simulink model "Fourteen_bus_simscape_V1o1"  (R2026a)
settings: Solver=ode23t  StopTime=12  FixedStep=0.2  RelTol=1e-2  AbsTol=1e-2  EnableMultiTasking=on
libraries: ee_lib x92, nesl_utility x64, fl_lib x25, eeRmsMeasurement x18, slpidlib x5, eeSmGovernor x2, elec_conv_HighZElecRef x1
(part 1 of 3)
settings Model: Creator=Bharath  LastModifiedBy=Mudassir
settings SolverCC: MaxConsecutiveMinStep=auto  ZeroCrossControl=DisableAll
settings DataIOCC: SignalLoggingSaveFormat=ModelDataLogs
settings DebuggingCC: SaveWithParameterizedLinksMsg=none  UnderspecifiedInitializationDetection=Classic
settings HardwareCC: ProdHWDeviceType=32-bit Generic
settings GRTTargetCC: CombineOutputUpdateFcns=off  GRTInterface=on
settings SimscapeCC: SimscapeNormalizeSystem=off  SimscapeLogType=none  SimscapeLogDataHistory=5000.0

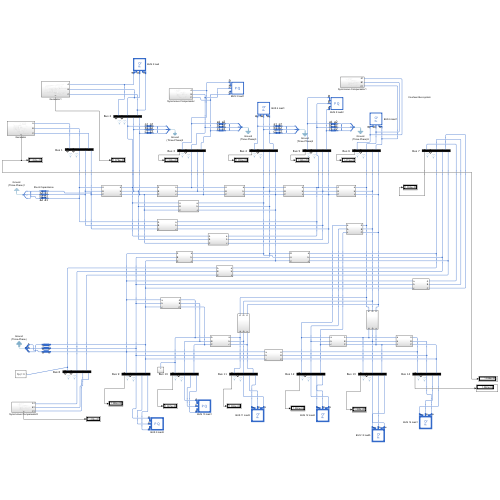
[thumbnail: Simulink's stored preview of the top-level diagram]
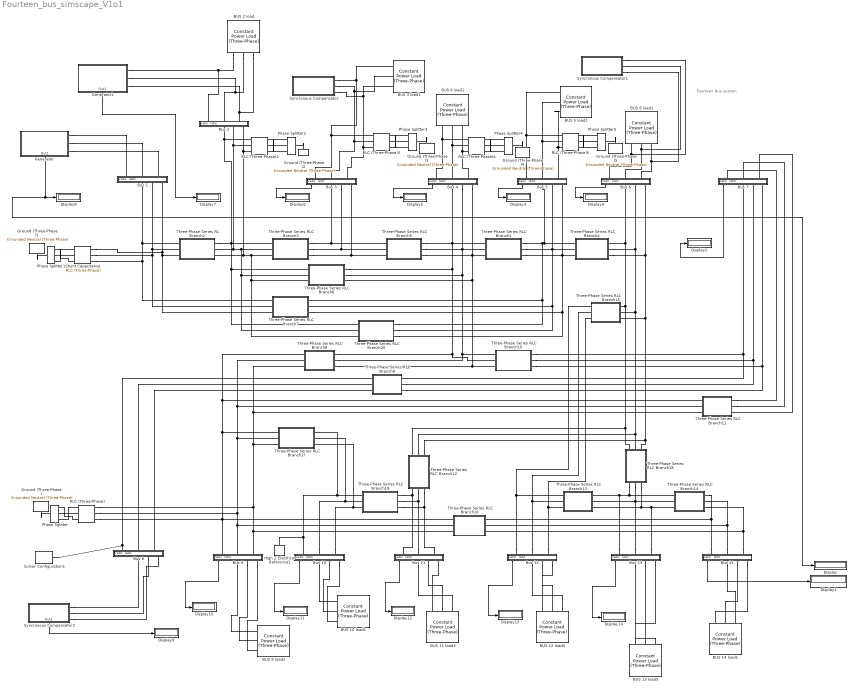
== system Fourteen_bus_simscape_V1o1 ==
  note: Fourteen Bus system
  BUS 10 load1 : ee_lib/Passive/Constant Power Load (Three-Phase)  port_option=ee.enum.threePhasePort.expanded  FRated=60 Hz  active_power=9.0e6 W  reactive_power=5.8e6 A*V  Vline_rms_min=92.4e3 V  tau=0.01 s  Vline_rms_ini=132e3 V  Vang_ini=0 deg  gmin=1e-6 S
  BUS 11 load3 : ee_lib/Passive/Constant Power Load (Three-Phase)  port_option=ee.enum.threePhasePort.expanded  FRated=60 Hz  active_power=3.5e6 W  reactive_power=1.8e6 A*V  Vline_rms_min=92.4e3 V  tau=0.01 s  Vline_rms_ini=132e3 V  Vang_ini=0 deg  gmin=1e-6 S
  BUS 12 load4 : ee_lib/Passive/Constant Power Load (Three-Phase)  port_option=ee.enum.threePhasePort.expanded  FRated=60 Hz  active_power=6.1e6 W  reactive_power=1.6e6 A*V  Vline_rms_min=92.4e3 V  tau=0.01 s  Vline_rms_ini=132e3 V  Vang_ini=0 deg  gmin=1e-6 S
  BUS 13 load5 : ee_lib/Passive/Constant Power Load (Three-Phase)  port_option=ee.enum.threePhasePort.expanded  FRated=60 Hz  active_power=13.5e6 W  reactive_power=5.8e6 A*V  Vline_rms_min=92.3e3 V  tau=0.01 s  Vline_rms_ini=132e3 V  Vang_ini=0 deg  gmin=1e-6 S
  BUS 14 load1 : ee_lib/Passive/Constant Power Load (Three-Phase)  port_option=ee.enum.threePhasePort.expanded  FRated=60 Hz  active_power=14.9e6 W  reactive_power=5.0e6 A*V  Vline_rms_min=92.4e3 V  tau=0.01 s  Vline_rms_ini=132e3 V  Vang_ini=0 deg  gmin=1e-6 S
  BUS 2 load : ee_lib/Passive/Constant Power Load (Three-Phase)  port_option=ee.enum.threePhasePort.expanded  FRated=60 Hz  active_power=21.7e6 W  reactive_power=12.7e6 A*V  Vline_rms_min=92.4 V  tau=0.01 s  Vline_rms_ini=132e3 V  Vang_ini=0 deg  gmin=1e-6 S
  BUS 3 load1 : ee_lib/Passive/Constant Power Load (Three-Phase)  port_option=ee.enum.threePhasePort.expanded  FRated=60 Hz  active_power=94.2e6 W  reactive_power=19.0e6 A*V  Vline_rms_min=92.4e3 V  tau=0.01 s  Vline_rms_ini=132e3 V  Vang_ini=0 deg  gmin=1e-6 S
  BUS 4 load1 : ee_lib/Passive/Constant Power Load (Three-Phase)  port_option=ee.enum.threePhasePort.expanded  FRated=60 Hz  active_power=47.8e6 W  reactive_power=-3.9e6 A*V  Vline_rms_min=92.4e3 V  tau=0.01 s  Vline_rms_ini=132e3 V  Vang_ini=0 deg  gmin=1e-6 S
  BUS 5 load2 : ee_lib/Passive/Constant Power Load (Three-Phase)  port_option=ee.enum.threePhasePort.expanded  FRated=60 Hz  active_power=7.6e6 W  reactive_power=1.6e6 A*V  Vline_rms_min=92.4e3 V  tau=0.01 s  Vline_rms_ini=132e3 V  Vang_ini=0 deg  gmin=1e-6 S
  BUS 6 load1 : ee_lib/Passive/Constant Power Load (Three-Phase)  port_option=ee.enum.threePhasePort.expanded  FRated=60 Hz  active_power=11.2e6 W  reactive_power=7.5e6 A*V  Vline_rms_min=92.4e3 V  tau=0.01 s  Vline_rms_ini=132e3 V  Vang_ini=0 deg  gmin=1e-6 S
  BUS 9 load2 : ee_lib/Passive/Constant Power Load (Three-Phase)  port_option=ee.enum.threePhasePort.expanded  FRated=60 Hz  active_power=29.5e6 W  reactive_power=16.6e6 A*V  Vline_rms_min=92.4e3 V  tau=0.01 s  Vline_rms_ini=132e3 V  Vang_ini=0 deg  gmin=1e-6 S
  "Bus 1 " : Subsystem
  "Bus 10 " : Subsystem
  "Bus 11 " : Subsystem
  "Bus 12 " : Subsystem
  "Bus 13 " : Subsystem
  "Bus 14 " : Subsystem
  "Bus 2 " : Subsystem
  "Bus 3 " : Subsystem
  "Bus 4 " : Subsystem
  "Bus 5 " : Subsystem
  "Bus 6 " : Subsystem
  "Bus 7 " : Subsystem
  "Bus 8 " : Subsystem
  "Bus 9 " : Subsystem
  Display{,1..14} (15 alike) : Display
  Generator : Subsystem
      settings: PortSchema="{\"entries\":[{\"content\":{\"sides\":[{\"content\":{},\"type\":\"ConnectorPlacement.EquallySpacedRectSide\",\"uuid\":\"dad8709b-30c0-4090-88e1-ec810a18cf3f\"},{\"content\":{\"connectorIds\":[\"RConn1\",\"RConn2\",\"RConn3\"],\"side\":\"RIGHT\"},\"type\":\"ConnectorPlacement.EquallySpacedRectSide\",\"uuid\":\"92b3fce1-089d-4b63-9622-725cf932acc2\"},{\"content\":{\"side\":\"TOP\"},\"type\":\"ConnectorPlacement.EquallySpacedRectSide\",\"uuid\":\"fda0afc2-97bc-4766-b49e-326dedc200bc\"},{\"content\":{\"connectorIds\":[\"Out1\"],\"side\":\"BOTTOM\"},\"type\":\"ConnectorPlacement.EquallySpacedRectSide\",\"uuid\":\"7b5f0a66-de7c-4105-acc6-abc867d9e61c\"}]},\"type\":\"ConnectorPlacement.EquallySpacedConnector\",\"uuid\":\"4ba6e797-8987-4af2-b0c1-b0b7a69cc685\"}],\"packageUris\":[\"http://schema.mathworks.com/mf0/Connector/R2020b\"],\"version\":\"1.0\"}"
  Generator1 : Subsystem
      settings: PortSchema="{\"entries\":[{\"content\":{\"sides\":[{\"content\":{},\"type\":\"ConnectorPlacement.EquallySpacedRectSide\",\"uuid\":\"dad8709b-30c0-4090-88e1-ec810a18cf3f\"},{\"content\":{\"connectorIds\":[\"RConn1\",\"RConn2\",\"RConn3\"],\"side\":\"RIGHT\"},\"type\":\"ConnectorPlacement.EquallySpacedRectSide\",\"uuid\":\"92b3fce1-089d-4b63-9622-725cf932acc2\"},{\"content\":{\"side\":\"TOP\"},\"type\":\"ConnectorPlacement.EquallySpacedRectSide\",\"uuid\":\"fda0afc2-97bc-4766-b49e-326dedc200bc\"},{\"content\":{\"connectorIds\":[\"Out1\"],\"side\":\"BOTTOM\"},\"type\":\"ConnectorPlacement.EquallySpacedRectSide\",\"uuid\":\"e381a1c8-2bd2-44ff-8304-e9f3baae7e4f\"}]},\"type\":\"ConnectorPlacement.EquallySpacedConnector\",\"uuid\":\"4ba6e797-8987-4af2-b0c1-b0b7a69cc685\"}],\"packageUris\":[\"http://schema.mathworks.com/mf0/Connector/R2020b\"],\"version\":\"1.0\"}"
  Ground (Three-Phase){,1..5} (6 alike) : ee_lib/Connectors & References/Grounded Neutral (Three-Phase)  port_option=ee.enum.threePhasePort.composite
  High Z Electrical Reference1 : elec_conv_HighZElecRef/High Z Electrical Reference  SystemSampleTime=-1  VariantActivationTime=update diagram  EmptyChoice=off  PassThrough=off  PassThroughVariantControl=(default)  EmptyChoiceVariantControl=(default)  AllowFlexibleInterface=on  Latency=0  AutoFrameSizeCalculation=off
  Phase Splitter{,1..5} (6 alike) : ee_lib/Connectors & References/Phase Splitter
  RLC (Three-Phase) : ee_lib/Passive/RLC Assemblies/RLC (Three-Phase)  port_option=ee.enum.threePhasePort.expanded  component_structure=ee.enum.rlc.structure.C  R=1 Ohm  L=1e-3 H  C=2.892e-6 F  R_parasitic=1 Ohm  G_parasitic=0 1/Ohm  IL_specify=off  IL_priority=High  IL=[0, 0, 0] A  IL_nominal_specify=off  IL_nominal_value=1  IL_nominal_unit=A  VC_specify=off  VC_priority=High  VC=[0, 0, 0] V  VC_nominal_specify=off  VC_nominal_value=1  VC_nominal_unit=V
  RLC (Three-Phase)2 : ee_lib/Passive/RLC Assemblies/RLC (Three-Phase)  port_option=ee.enum.threePhasePort.expanded  component_structure=ee.enum.rlc.structure.C  R=1 Ohm  L=1e-3 H  C=1.257e-6 F  R_parasitic=1 Ohm  G_parasitic=0 1/Ohm  IL_specify=off  IL_priority=High  IL=[0, 0, 0] A  IL_nominal_specify=off  IL_nominal_value=1  IL_nominal_unit=A  VC_specify=off  VC_priority=High  VC=[0, 0, 0] V  VC_nominal_specify=off  VC_nominal_value=1  VC_nominal_unit=V
  RLC (Three-Phase)3 : ee_lib/Passive/RLC Assemblies/RLC (Three-Phase)  port_option=ee.enum.threePhasePort.expanded  component_structure=ee.enum.rlc.structure.C  R=1 Ohm  L=1e-3 H  C=5.922e-7 F  R_parasitic=1 Ohm  G_parasitic=0 1/Ohm  IL_specify=off  IL_priority=High  IL=[0, 0, 0] A  IL_nominal_specify=off  IL_nominal_value=1  IL_nominal_unit=A  VC_specify=off  VC_priority=High  VC=[0, 0, 0] V  VC_nominal_specify=off  VC_nominal_value=1  VC_nominal_unit=V
  RLC (Three-Phase)4 : ee_lib/Passive/RLC Assemblies/RLC (Three-Phase)  port_option=ee.enum.threePhasePort.expanded  component_structure=ee.enum.rlc.structure.C  R=1 Ohm  L=1e-3 H  C=5.176e-7 F  R_parasitic=1 Ohm  G_parasitic=0 1/Ohm  IL_specify=off  IL_priority=High  IL=[0, 0, 0] A  IL_nominal_specify=off  IL_nominal_value=1  IL_nominal_unit=A  VC_specify=off  VC_priority=High  VC=[0, 0, 0] V  VC_nominal_specify=off  VC_nominal_value=1  VC_nominal_unit=V
  RLC (Three-Phase)5 : ee_lib/Passive/RLC Assemblies/RLC (Three-Phase)  port_option=ee.enum.threePhasePort.expanded  component_structure=ee.enum.rlc.structure.C  R=1 Ohm  L=1e-3 H  C=6.493e-7 F  R_parasitic=1 Ohm  G_parasitic=0 1/Ohm  IL_specify=off  IL_priority=High  IL=[0, 0, 0] A  IL_nominal_specify=off  IL_nominal_value=1  IL_nominal_unit=A  VC_specify=off  VC_priority=High  VC=[0, 0, 0] V  VC_nominal_specify=off  VC_nominal_value=1  VC_nominal_unit=V
  Shunt Capacitance : ee_lib/Passive/RLC Assemblies/RLC (Three-Phase)  port_option=ee.enum.threePhasePort.expanded  component_structure=ee.enum.rlc.structure.C  R=1 Ohm  L=1e-3 H  C=7.878e-7 F  R_parasitic=1 Ohm  G_parasitic=0 1/Ohm  IL_specify=off  IL_priority=High  IL=[0, 0, 0] A  IL_nominal_specify=off  IL_nominal_value=1  IL_nominal_unit=A  VC_specify=off  VC_priority=High  VC=[0, 0, 0] V  VC_nominal_specify=off  VC_nominal_value=1  VC_nominal_unit=V
  Solver Configuration1 : nesl_utility/Solver Configuration  PhysicalDomain=network_engine_domain  SubClassName=solver  LeftPortType=input  RightPortType=generic  Tones=[]  Harmonics=[]  SimulateNoise=off  Profile=off  UseLocalSampling=off  EnableSwitchedLinearOptims=on  FrequencyDomain=off  UseCCode=off  RelTol=0.001  AbsTol=0.001  MinStep=1e-09  ToWorkspace=off  RevertToSquareIcSolve=off  NumHomotopyIterations=100  PhasorMode=off  PhasorModeNumHarmonics=1  ConsistencySolver=NEWTON_XTOL_AFTER_FTOL  CanonicalOrdering=CANONICAL  OptimizeIntermediates=OPTIMIZED  IndexReductionMethod=DerivativeReplacement  DoDC=off  ResidualTolerance=1e-09  ConsistencyTolSource=GLOBAL  ConsistencyAbsTol=0.001  ConsistencyRelTol=0.001  ConsistencyTolFactor=0.001  UseLocalSolver=off  LocalSolverChoice=NE_BACKWARD_EULER_ADVANCER  ResolveIndetEquations=on  FunctionEvalNumThread=1  LocalSolverSampleTime=0.001  DoFixedCost=off  MaxNonlinIter=3  MaxModeIter=2  ComputeImpulses=off  ImpulseIterations=2  LinearAlgebra=auto  LinearAlgebraNumThread=0  EquationFormulation=NE_TIME_EF  DelaysMemoryBudget=1024  AutomaticFiltering=on  FilteringTimeConstant=0.001  PartitionStorageMethod=AS_NEEDED  PartitionMemoryBudget=1024  PartitionMethod=ROBUST  MultibodyUseLocalSolver=off  MultibodyLocalSolverChoice=ODE1  MultibodyLocalSolverSampleTime=0.001
  Syncronous Compensator : Subsystem
  Syncronous Compensator1 : Subsystem
  Syncronous Compensator2 : Subsystem
      settings: PortSchema="{\"entries\":[{\"content\":{\"sides\":[{\"content\":{},\"type\":\"ConnectorPlacement.EquallySpacedRectSide\",\"uuid\":\"dad8709b-30c0-4090-88e1-ec810a18cf3f\"},{\"content\":{\"connectorIds\":[\"RConn1\",\"RConn2\",\"RConn3\"],\"side\":\"RIGHT\"},\"type\":\"ConnectorPlacement.EquallySpacedRectSide\",\"uuid\":\"92b3fce1-089d-4b63-9622-725cf932acc2\"},{\"content\":{\"side\":\"TOP\"},\"type\":\"ConnectorPlacement.EquallySpacedRectSide\",\"uuid\":\"fda0afc2-97bc-4766-b49e-326dedc200bc\"},{\"content\":{\"connectorIds\":[\"Out1\"],\"side\":\"BOTTOM\"},\"type\":\"ConnectorPlacement.EquallySpacedRectSide\",\"uuid\":\"87e71bf6-f82f-4acd-82d9-e7a3dc4e74e7\"}]},\"type\":\"ConnectorPlacement.EquallySpacedConnector\",\"uuid\":\"4ba6e797-8987-4af2-b0c1-b0b7a69cc685\"}],\"packageUris\":[\"http://schema.mathworks.com/mf0/Connector/R2020b\"],\"version\":\"1.0\"}"
  Three-Phase Series RL Branch2 : Subsystem
      settings: AttributesFormatString=\n
  Three-Phase Series RLC Branch1 : Subsystem
      settings: AttributesFormatString=\n
  Three-Phase Series RLC Branch10 : Subsystem
      settings: AttributesFormatString=\n
  Three-Phase Series RLC Branch11 : Subsystem
      settings: AttributesFormatString=\n
  Three-Phase Series RLC Branch12 : Subsystem
      settings: AttributesFormatString=\n
  Three-Phase Series RLC Branch13 : Subsystem
      settings: AttributesFormatString=\n
  Three-Phase Series RLC Branch14 : Subsystem
      settings: AttributesFormatString=\n
  Three-Phase Series RLC Branch15 : Subsystem
      settings: AttributesFormatString=\n
  Three-Phase Series RLC Branch16 : Subsystem
      settings: AttributesFormatString=\n
  Three-Phase Series RLC Branch17 : Subsystem
      settings: AttributesFormatString=\n
  Three-Phase Series RLC Branch18 : Subsystem
      settings: AttributesFormatString=\n
  Three-Phase Series RLC Branch19 : Subsystem
      settings: AttributesFormatString=\n
  Three-Phase Series RLC Branch20 : Subsystem
      settings: AttributesFormatString=\n
  Three-Phase Series RLC Branch3 : Subsystem
      settings: AttributesFormatString=\n
  Three-Phase Series RLC Branch4 : Subsystem
      settings: AttributesFormatString=\n
  Three-Phase Series RLC Branch5 : Subsystem
      settings: AttributesFormatString=\n
  Three-Phase Series RLC Branch6 : Subsystem
      settings: AttributesFormatString=\n
  Three-Phase Series RLC Branch7 : Subsystem
      settings: AttributesFormatString=\n
  Three-Phase Series RLC Branch8 : Subsystem
      settings: AttributesFormatString=\n
  Three-Phase Series RLC Branch9 : Subsystem
      settings: AttributesFormatString=\n
  wires:
  "Bus 7 "/1(Vabc) -> Display2/1
  "Bus 5 "/1(Vabc) -> Display3/1
  "Bus 6 "/1(Vabc) -> Display4/1
  "Bus 4 "/1(Vabc) -> Display5/1
  "Bus 3 "/1(Vabc) -> Display6/1
  Generator1/1(Out1) -> Display7/1
  Generator/1(Out1) -> Display/1, Display8/1
  Syncronous Compensator2/1(Out1) -> Display9/1
  "Bus 9 "/1(Vabc) -> Display10/1
  "Bus 10 "/1(Vabc) -> Display11/1
  "Bus 11 "/1(Vabc) -> Display12/1
  "Bus 12 "/1(Vabc) -> Display13/1
  "Bus 13 "/1(Vabc) -> Display14/1
  "Bus 14 "/1(Vabc) -> Display1/1
  connections:
  "Bus 9 "/LConn3 -- Three-Phase Series RLC Branch16/RConn3 -- RLC (Three-Phase)/LConn3 -- Three-Phase Series RLC Branch17/RConn3 -- Three-Phase Series RLC Branch11/RConn3 -- Three-Phase Series RLC Branch8/LConn3
  "Bus 9 "/LConn2 -- Three-Phase Series RLC Branch16/RConn2 -- RLC (Three-Phase)/LConn2 -- Three-Phase Series RLC Branch17/RConn2 -- Three-Phase Series RLC Branch11/RConn2 -- Three-Phase Series RLC Branch8/LConn2
  "Bus 9 "/LConn1 -- RLC (Three-Phase)/LConn1 -- Three-Phase Series RLC Branch16/RConn1 -- Three-Phase Series RLC Branch17/RConn1 -- Three-Phase Series RLC Branch11/RConn1 -- Three-Phase Series RLC Branch8/LConn1
  "Bus 7 "/RConn3 -- Three-Phase Series RLC Branch10/RConn3 -- Three-Phase Series RLC Branch9/RConn3
  "Bus 7 "/RConn2 -- Three-Phase Series RLC Branch10/RConn2 -- Three-Phase Series RLC Branch9/RConn2
  "Bus 7 "/RConn1 -- Three-Phase Series RLC Branch10/RConn1 -- Three-Phase Series RLC Branch9/RConn1
  "Bus 6 "/RConn3 -- Three-Phase Series RLC Branch4/RConn3 -- Three-Phase Series RLC Branch18/LConn3 -- Three-Phase Series RLC Branch12/LConn3 -- Three-Phase Series RLC Branch15/LConn3
  "Bus 6 "/RConn2 -- Three-Phase Series RLC Branch15/LConn2 -- Three-Phase Series RLC Branch18/LConn2 -- Three-Phase Series RLC Branch12/LConn2 -- Three-Phase Series RLC Branch4/RConn2
  "Bus 6 "/RConn1 -- Three-Phase Series RLC Branch18/LConn1 -- Three-Phase Series RLC Branch12/LConn1 -- Three-Phase Series RLC Branch15/LConn1 -- Three-Phase Series RLC Branch4/RConn1
  "Bus 5 "/RConn3 -- Three-Phase Series RLC Branch1/RConn3 -- Three-Phase Series RLC Branch20/RConn3 -- Three-Phase Series RLC Branch7/RConn3 -- Three-Phase Series RLC Branch4/LConn3
  "Bus 5 "/RConn2 -- Three-Phase Series RLC Branch1/RConn2 -- Three-Phase Series RLC Branch20/RConn2 -- Three-Phase Series RLC Branch7/RConn2 -- Three-Phase Series RLC Branch4/LConn2
  "Bus 5 "/RConn1 -- Three-Phase Series RLC Branch1/RConn1 -- Three-Phase Series RLC Branch20/RConn1 -- Three-Phase Series RLC Branch7/RConn1 -- Three-Phase Series RLC Branch4/LConn1
  "Bus 3 "/RConn2 -- Three-Phase Series RLC Branch5/LConn2 -- Three-Phase Series RLC Branch3/RConn2
  "Bus 3 "/RConn1 -- Three-Phase Series RLC Branch5/LConn1 -- Three-Phase Series RLC Branch3/RConn1
  Three-Phase Series RLC Branch20/LConn3 -- Three-Phase Series RLC Branch6/LConn3 -- Three-Phase Series RLC Branch3/LConn3 -- Three-Phase Series RL Branch2/RConn3 -- RLC (Three-Phase)2/LConn3 -- "Bus 2 "/RConn3
  Three-Phase Series RLC Branch3/LConn2 -- Three-Phase Series RLC Branch20/LConn2 -- Three-Phase Series RLC Branch6/LConn2 -- Three-Phase Series RL Branch2/RConn2 -- RLC (Three-Phase)2/LConn2 -- "Bus 2 "/RConn2
  Three-Phase Series RLC Branch3/LConn1 -- Three-Phase Series RLC Branch20/LConn1 -- Three-Phase Series RLC Branch6/LConn1 -- Three-Phase Series RL Branch2/RConn1 -- RLC (Three-Phase)2/LConn1 -- "Bus 2 "/RConn1
  BUS 2 load/LConn2 -- Generator1/RConn2 -- "Bus 2 "/LConn2
  BUS 2 load/LConn1 -- Generator1/RConn1 -- "Bus 2 "/LConn1
  "Bus 14 "/LConn3 -- Three-Phase Series RLC Branch14/LConn3 -- Three-Phase Series RLC Branch16/LConn3
  "Bus 14 "/LConn2 -- Three-Phase Series RLC Branch14/LConn2 -- Three-Phase Series RLC Branch16/LConn2
  "Bus 14 "/LConn1 -- Three-Phase Series RLC Branch14/LConn1 -- Three-Phase Series RLC Branch16/LConn1
  "Bus 13 "/LConn3 -- Three-Phase Series RLC Branch18/RConn3 -- Three-Phase Series RLC Branch13/LConn3 -- Three-Phase Series RLC Branch14/RConn3
  "Bus 13 "/LConn2 -- Three-Phase Series RLC Branch18/RConn2 -- Three-Phase Series RLC Branch14/RConn2 -- Three-Phase Series RLC Branch13/LConn2
  "Bus 13 "/LConn1 -- Three-Phase Series RLC Branch18/RConn1 -- Three-Phase Series RLC Branch14/RConn1 -- Three-Phase Series RLC Branch13/LConn1
  "Bus 12 "/LConn3 -- Three-Phase Series RLC Branch13/RConn3 -- Three-Phase Series RLC Branch15/RConn3
  "Bus 12 "/LConn2 -- Three-Phase Series RLC Branch13/RConn2 -- Three-Phase Series RLC Branch15/RConn2
  "Bus 12 "/LConn1 -- Three-Phase Series RLC Branch13/RConn1 -- Three-Phase Series RLC Branch15/RConn1
  "Bus 11 "/LConn3 -- Three-Phase Series RLC Branch12/RConn3 -- Three-Phase Series RLC Branch19/RConn3
  "Bus 11 "/LConn2 -- Three-Phase Series RLC Branch12/RConn2 -- Three-Phase Series RLC Branch19/RConn2
  "Bus 11 "/LConn1 -- Three-Phase Series RLC Branch12/RConn1 -- Three-Phase Series RLC Branch19/RConn1
  "Bus 10 "/LConn3 -- Three-Phase Series RLC Branch17/LConn3 -- Three-Phase Series RLC Branch19/LConn3
  "Bus 10 "/LConn2 -- Three-Phase Series RLC Branch17/LConn2 -- Three-Phase Series RLC Branch19/LConn2
  Three-Phase Series RLC Branch17/LConn1 -- Three-Phase Series RLC Branch19/LConn1 -- "Bus 10 "/LConn1 -- High Z Electrical Reference1/LConn1
  Three-Phase Series RL Branch2/LConn3 -- Three-Phase Series RLC Branch7/LConn3 -- "Bus 1 "/RConn3 -- Shunt Capacitance/LConn3
  "Bus 1 "/RConn2 -- Three-Phase Series RL Branch2/LConn2 -- Shunt Capacitance/LConn2 -- Three-Phase Series RLC Branch7/LConn2
  "Bus 1 "/RConn1 -- Three-Phase Series RL Branch2/LConn1 -- Shunt Capacitance/LConn1 -- Three-Phase Series RLC Branch7/LConn1
  "Bus 4 "/LConn3 -- RLC (Three-Phase)4/LConn3 -- BUS 4 load1/LConn3
  Syncronous Compensator2/RConn3 -- "Bus 8 "/RConn3
  Syncronous Compensator2/RConn2 -- "Bus 8 "/RConn2
  Syncronous Compensator2/RConn1 -- "Bus 8 "/RConn1
  "Bus 9 "/RConn2 -- BUS 9 load2/LConn2
  "Bus 9 "/RConn1 -- BUS 9 load2/LConn1
  "Bus 9 "/RConn3 -- BUS 9 load2/LConn3
  "Bus 4 "/LConn2 -- RLC (Three-Phase)4/LConn2 -- BUS 4 load1/LConn2
  BUS 5 load2/LConn1 -- RLC (Three-Phase)5/LConn1 -- "Bus 5 "/LConn1
  BUS 5 load2/LConn3 -- RLC (Three-Phase)5/LConn3 -- "Bus 5 "/LConn3
  "Bus 7 "/LConn3 -- Three-Phase Series RLC Branch11/LConn3
  BUS 5 load2/LConn2 -- "Bus 5 "/LConn2 -- RLC (Three-Phase)5/LConn2
  "Bus 14 "/RConn3 -- BUS 14 load1/LConn3
  "Bus 14 "/RConn2 -- BUS 14 load1/LConn2
  "Bus 14 "/RConn1 -- BUS 14 load1/LConn1
  "Bus 13 "/RConn3 -- BUS 13 load5/LConn3
  "Bus 13 "/RConn2 -- BUS 13 load5/LConn2
  "Bus 13 "/RConn1 -- BUS 13 load5/LConn1
  "Bus 12 "/RConn3 -- BUS 12 load4/LConn3
  "Bus 12 "/RConn2 -- BUS 12 load4/LConn2
  "Bus 12 "/RConn1 -- BUS 12 load4/LConn1
  "Bus 11 "/RConn3 -- BUS 11 load3/LConn3
  "Bus 11 "/RConn2 -- BUS 11 load3/LConn2
  "Bus 11 "/RConn1 -- BUS 11 load3/LConn1
  "Bus 10 "/RConn3 -- BUS 10 load1/LConn3
  "Bus 10 "/RConn2 -- BUS 10 load1/LConn2
  "Bus 10 "/RConn1 -- BUS 10 load1/LConn1
  BUS 2 load/LConn3 -- Generator1/RConn3 -- "Bus 2 "/LConn3
  "Bus 8 "/LConn1 -- Three-Phase Series RLC Branch9/LConn1 -- Solver Configuration1/RConn1
  Three-Phase Series RLC Branch9/LConn2 -- "Bus 8 "/LConn2
  Three-Phase Series RLC Branch9/LConn3 -- "Bus 8 "/LConn3
  "Bus 4 "/LConn1 -- RLC (Three-Phase)4/LConn1 -- BUS 4 load1/LConn1
  Three-Phase Series RLC Branch11/LConn2 -- "Bus 7 "/LConn2
  Three-Phase Series RLC Branch11/LConn1 -- "Bus 7 "/LConn1
  Syncronous Compensator/RConn2 -- BUS 3 load1/LConn2 -- "Bus 3 "/LConn2 -- RLC (Three-Phase)3/LConn2
  Syncronous Compensator/RConn1 -- BUS 3 load1/LConn1 -- RLC (Three-Phase)3/LConn1 -- "Bus 3 "/LConn1
  Syncronous Compensator/RConn3 -- BUS 3 load1/LConn3 -- RLC (Three-Phase)3/LConn3 -- "Bus 3 "/LConn3
  "Bus 6 "/LConn2 -- Syncronous Compensator1/RConn2 -- BUS 6 load1/LConn2
  "Bus 6 "/LConn1 -- Syncronous Compensator1/RConn1 -- BUS 6 load1/LConn1
  "Bus 6 "/LConn3 -- Syncronous Compensator1/RConn3 -- BUS 6 load1/LConn3
  "Bus 4 "/RConn3 -- Three-Phase Series RLC Branch1/LConn3 -- Three-Phase Series RLC Branch5/RConn3 -- Three-Phase Series RLC Branch6/RConn3 -- Three-Phase Series RLC Branch10/LConn3 -- Three-Phase Series RLC Branch8/RConn3
  "Bus 4 "/RConn2 -- Three-Phase Series RLC Branch1/LConn2 -- Three-Phase Series RLC Branch6/RConn2 -- Three-Phase Series RLC Branch8/RConn2 -- Three-Phase Series RLC Branch10/LConn1 -- Three-Phase Series RLC Branch5/RConn2
  "Bus 4 "/RConn1 -- Three-Phase Series RLC Branch1/LConn1 -- Three-Phase Series RLC Branch6/RConn1 -- Three-Phase Series RLC Branch10/LConn2 -- Three-Phase Series RLC Branch8/RConn1 -- Three-Phase Series RLC Branch5/RConn1
  "Bus 3 "/RConn3 -- Three-Phase Series RLC Branch5/LConn3 -- Three-Phase Series RLC Branch3/RConn3
  Generator/RConn3 -- "Bus 1 "/LConn3
  Generator/RConn1 -- "Bus 1 "/LConn1
  Generator/RConn2 -- "Bus 1 "/LConn2
  Ground (Three-Phase)/LConn1 -- Phase Splitter/LConn1
  RLC (Three-Phase)/RConn3 -- Phase Splitter/RConn3
  RLC (Three-Phase)/RConn2 -- Phase Splitter/RConn2
  RLC (Three-Phase)/RConn1 -- Phase Splitter/RConn1
  Shunt Capacitance/RConn1 -- Phase Splitter1/RConn1
  Ground (Three-Phase)1/LConn1 -- Phase Splitter1/LConn1
  Shunt Capacitance/RConn3 -- Phase Splitter1/RConn3
  Shunt Capacitance/RConn2 -- Phase Splitter1/RConn2
  RLC (Three-Phase)2/RConn3 -- Phase Splitter2/RConn3
  RLC (Three-Phase)2/RConn2 -- Phase Splitter2/RConn2
  Ground (Three-Phase)2/LConn1 -- Phase Splitter2/LConn1
  RLC (Three-Phase)2/RConn1 -- Phase Splitter2/RConn1
  RLC (Three-Phase)3/RConn3 -- Phase Splitter3/RConn3
  RLC (Three-Phase)3/RConn2 -- Phase Splitter3/RConn2
  Ground (Three-Phase)3/LConn1 -- Phase Splitter3/LConn1
  RLC (Three-Phase)3/RConn1 -- Phase Splitter3/RConn1
  RLC (Three-Phase)4/RConn3 -- Phase Splitter4/RConn3
  RLC (Three-Phase)4/RConn2 -- Phase Splitter4/RConn2
  Ground (Three-Phase)4/LConn1 -- Phase Splitter4/LConn1
  RLC (Three-Phase)4/RConn1 -- Phase Splitter4/RConn1
  RLC (Three-Phase)5/RConn3 -- Phase Splitter5/RConn3
  RLC (Three-Phase)5/RConn2 -- Phase Splitter5/RConn2
  Ground (Three-Phase)5/LConn1 -- Phase Splitter5/LConn1
  RLC (Three-Phase)5/RConn1 -- Phase Splitter5/RConn1

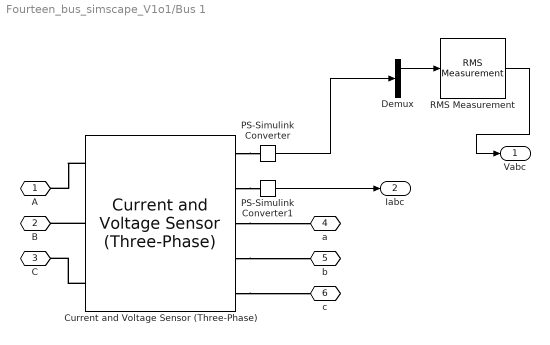
== system Fourteen_bus_simscape_V1o1/Bus 1  ==
  Current and Voltage Sensor (Three-Phase) : ee_lib/Sensors & Transducers/Current and Voltage Sensor (Three-Phase)  port_option=ee.enum.threePhasePort.expanded  vMeasurementType=ee.enum.vmeasurement.ll  outputUnit=ee.enum.unit.si  SRated=100000000 V*A  VRated=0.95 V  I_specify=off  I_priority=None  I=[ 0 0 0 ] A  I_nominal_specify=off  I_nominal_value=1  I_nominal_unit=A  V_specify=off  V_priority=None  V=[ 0 0 0 ] V  V_nominal_specify=off  V_nominal_value=1  V_nominal_unit=V
  Demux : Demux  Outputs=3
  PS-Simulink Converter : nesl_utility/PS-Simulink Converter  PhysicalDomain=network_engine_domain  SubClassName=ps_output  LeftPortType=input  RightPortType=output  PseudoPeriodic=off  Frequencies=[]  VectorFormat=1-D array  Unit=1  AffineConversion=off
  PS-Simulink Converter1 : nesl_utility/PS-Simulink Converter  PhysicalDomain=network_engine_domain  SubClassName=ps_output  LeftPortType=input  RightPortType=output  PseudoPeriodic=off  Frequencies=[]  VectorFormat=1-D array  Unit=1  AffineConversion=off
  RMS Measurement : eeRmsMeasurement/RMS Measurement  LabelModeActiveChoice=Total  F=60  SpecifyHarmonics=off  K=[0 1 2]  Ts=0
      settings: LibrarySourceBlock=|
      | ee_sl_lib/Measurements/RMS
      | Measurement
  A : PMIOPort  Side=Left
  B : PMIOPort  Port=2  Side=Left
  C : PMIOPort  Port=3  Side=Left
  a : PMIOPort  Port=4  Side=Right
  b : PMIOPort  Port=5  Side=Right
  c : PMIOPort  Port=6  Side=Right
  Vabc : Outport  VectorParamsAs1DForOutWhenUnconnected=off
  Iabc : Outport  Port=2  VectorParamsAs1DForOutWhenUnconnected=off
  wires:
  PS-Simulink Converter1/1 -> Iabc/1
  RMS Measurement/1 -> Vabc/1
  Demux/1 -> RMS Measurement/1
  PS-Simulink Converter/1 -> Demux/1
  connections:
  Current and Voltage Sensor (Three-Phase)/RConn1 -- PS-Simulink Converter/LConn1
  Current and Voltage Sensor (Three-Phase)/RConn2 -- PS-Simulink Converter1/LConn1
  Current and Voltage Sensor (Three-Phase)/RConn5 -- c/RConn1
  Current and Voltage Sensor (Three-Phase)/RConn4 -- b/RConn1
  Current and Voltage Sensor (Three-Phase)/RConn3 -- a/RConn1
  Current and Voltage Sensor (Three-Phase)/LConn3 -- C/RConn1
  Current and Voltage Sensor (Three-Phase)/LConn1 -- A/RConn1
  Current and Voltage Sensor (Three-Phase)/LConn2 -- B/RConn1

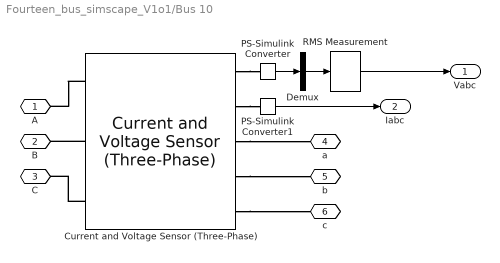
== system Fourteen_bus_simscape_V1o1/Bus 10  ==
  Current and Voltage Sensor (Three-Phase) : ee_lib/Sensors & Transducers/Current and Voltage Sensor (Three-Phase)  port_option=ee.enum.threePhasePort.expanded  vMeasurementType=ee.enum.vmeasurement.ll  outputUnit=ee.enum.unit.si  SRated=100000000 V*A  VRated=0.94 V  I_specify=off  I_priority=None  I=[ 0 0 0 ] A  I_nominal_specify=off  I_nominal_value=1  I_nominal_unit=A  V_specify=off  V_priority=None  V=[ 0 0 0 ] V  V_nominal_specify=off  V_nominal_value=1  V_nominal_unit=V
  Demux : Demux  Outputs=3
  PS-Simulink Converter : nesl_utility/PS-Simulink Converter  PhysicalDomain=network_engine_domain  SubClassName=ps_output  LeftPortType=input  RightPortType=output  PseudoPeriodic=off  Frequencies=[]  VectorFormat=1-D array  Unit=1  AffineConversion=off
  PS-Simulink Converter1 : nesl_utility/PS-Simulink Converter  PhysicalDomain=network_engine_domain  SubClassName=ps_output  LeftPortType=input  RightPortType=output  PseudoPeriodic=off  Frequencies=[]  VectorFormat=1-D array  Unit=1  AffineConversion=off
  RMS Measurement : eeRmsMeasurement/RMS Measurement  LabelModeActiveChoice=Total  F=60  SpecifyHarmonics=off  K=[0 1 2]  Ts=0
      settings: LibrarySourceBlock=|
      | ee_sl_lib/Measurements/RMS
      | Measurement
  A : PMIOPort  Side=Left
  B : PMIOPort  Port=2  Side=Left
  C : PMIOPort  Port=3  Side=Left
  a : PMIOPort  Port=4  Side=Right
  b : PMIOPort  Port=5  Side=Right
  c : PMIOPort  Port=6  Side=Right
  Vabc : Outport  VectorParamsAs1DForOutWhenUnconnected=off
  Iabc : Outport  Port=2  VectorParamsAs1DForOutWhenUnconnected=off
  wires:
  PS-Simulink Converter1/1 -> Iabc/1
  Demux/2 -> RMS Measurement/1
  RMS Measurement/1 -> Vabc/1
  PS-Simulink Converter/1 -> Demux/1
  connections:
  Current and Voltage Sensor (Three-Phase)/RConn1 -- PS-Simulink Converter/LConn1
  Current and Voltage Sensor (Three-Phase)/RConn2 -- PS-Simulink Converter1/LConn1
  Current and Voltage Sensor (Three-Phase)/RConn5 -- c/RConn1
  Current and Voltage Sensor (Three-Phase)/RConn4 -- b/RConn1
  Current and Voltage Sensor (Three-Phase)/RConn3 -- a/RConn1
  Current and Voltage Sensor (Three-Phase)/LConn3 -- C/RConn1
  Current and Voltage Sensor (Three-Phase)/LConn1 -- A/RConn1
  Current and Voltage Sensor (Three-Phase)/LConn2 -- B/RConn1

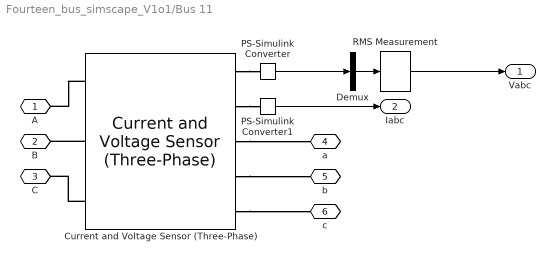
== system Fourteen_bus_simscape_V1o1/Bus 11  ==
  Current and Voltage Sensor (Three-Phase) : ee_lib/Sensors & Transducers/Current and Voltage Sensor (Three-Phase)  port_option=ee.enum.threePhasePort.expanded  vMeasurementType=ee.enum.vmeasurement.ll  outputUnit=ee.enum.unit.si  SRated=100000000 V*A  VRated=0.95 V  I_specify=off  I_priority=None  I=[ 0 0 0 ] A  I_nominal_specify=off  I_nominal_value=1  I_nominal_unit=A  V_specify=off  V_priority=None  V=[ 0 0 0 ] V  V_nominal_specify=off  V_nominal_value=1  V_nominal_unit=V
  Demux : Demux  Outputs=3
  PS-Simulink Converter : nesl_utility/PS-Simulink Converter  PhysicalDomain=network_engine_domain  SubClassName=ps_output  LeftPortType=input  RightPortType=output  PseudoPeriodic=off  Frequencies=[]  VectorFormat=1-D array  Unit=1  AffineConversion=off
  PS-Simulink Converter1 : nesl_utility/PS-Simulink Converter  PhysicalDomain=network_engine_domain  SubClassName=ps_output  LeftPortType=input  RightPortType=output  PseudoPeriodic=off  Frequencies=[]  VectorFormat=1-D array  Unit=1  AffineConversion=off
  RMS Measurement : eeRmsMeasurement/RMS Measurement  LabelModeActiveChoice=Total  F=60  SpecifyHarmonics=off  K=[0 1 2]  Ts=0
      settings: LibrarySourceBlock=|
      | ee_sl_lib/Measurements/RMS
      | Measurement
  A : PMIOPort  Side=Left
  B : PMIOPort  Port=2  Side=Left
  C : PMIOPort  Port=3  Side=Left
  a : PMIOPort  Port=4  Side=Right
  b : PMIOPort  Port=5  Side=Right
  c : PMIOPort  Port=6  Side=Right
  Vabc : Outport  VectorParamsAs1DForOutWhenUnconnected=off
  Iabc : Outport  Port=2  VectorParamsAs1DForOutWhenUnconnected=off
  wires:
  PS-Simulink Converter1/1 -> Iabc/1
  Demux/2 -> RMS Measurement/1
  PS-Simulink Converter/1 -> Demux/1
  RMS Measurement/1 -> Vabc/1
  connections:
  Current and Voltage Sensor (Three-Phase)/RConn1 -- PS-Simulink Converter/LConn1
  Current and Voltage Sensor (Three-Phase)/RConn2 -- PS-Simulink Converter1/LConn1
  Current and Voltage Sensor (Three-Phase)/RConn5 -- c/RConn1
  Current and Voltage Sensor (Three-Phase)/RConn4 -- b/RConn1
  Current and Voltage Sensor (Three-Phase)/RConn3 -- a/RConn1
  Current and Voltage Sensor (Three-Phase)/LConn3 -- C/RConn1
  Current and Voltage Sensor (Three-Phase)/LConn1 -- A/RConn1
  Current and Voltage Sensor (Three-Phase)/LConn2 -- B/RConn1

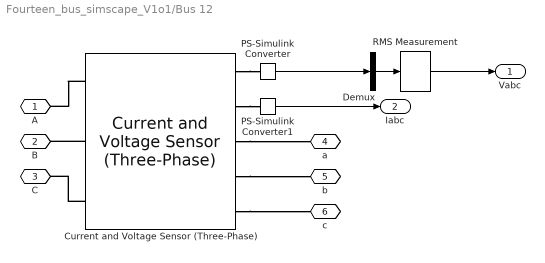
== system Fourteen_bus_simscape_V1o1/Bus 12  ==
  Current and Voltage Sensor (Three-Phase) : ee_lib/Sensors & Transducers/Current and Voltage Sensor (Three-Phase)  port_option=ee.enum.threePhasePort.expanded  vMeasurementType=ee.enum.vmeasurement.ll  outputUnit=ee.enum.unit.si  SRated=100000000 V*A  VRated=0.95 V  I_specify=off  I_priority=None  I=[ 0 0 0 ] A  I_nominal_specify=off  I_nominal_value=1  I_nominal_unit=A  V_specify=off  V_priority=None  V=[ 0 0 0 ] V  V_nominal_specify=off  V_nominal_value=1  V_nominal_unit=V
  Demux : Demux  Outputs=3
  PS-Simulink Converter : nesl_utility/PS-Simulink Converter  PhysicalDomain=network_engine_domain  SubClassName=ps_output  LeftPortType=input  RightPortType=output  PseudoPeriodic=off  Frequencies=[]  VectorFormat=1-D array  Unit=1  AffineConversion=off
  PS-Simulink Converter1 : nesl_utility/PS-Simulink Converter  PhysicalDomain=network_engine_domain  SubClassName=ps_output  LeftPortType=input  RightPortType=output  PseudoPeriodic=off  Frequencies=[]  VectorFormat=1-D array  Unit=1  AffineConversion=off
  RMS Measurement : eeRmsMeasurement/RMS Measurement  LabelModeActiveChoice=Total  F=60  SpecifyHarmonics=off  K=[0 1 2]  Ts=0
      settings: LibrarySourceBlock=|
      | ee_sl_lib/Measurements/RMS
      | Measurement
  A : PMIOPort  Side=Left
  B : PMIOPort  Port=2  Side=Left
  C : PMIOPort  Port=3  Side=Left
  a : PMIOPort  Port=4  Side=Right
  b : PMIOPort  Port=5  Side=Right
  c : PMIOPort  Port=6  Side=Right
  Vabc : Outport  VectorParamsAs1DForOutWhenUnconnected=off
  Iabc : Outport  Port=2  VectorParamsAs1DForOutWhenUnconnected=off
  wires:
  PS-Simulink Converter1/1 -> Iabc/1
  Demux/2 -> RMS Measurement/1
  PS-Simulink Converter/1 -> Demux/1
  RMS Measurement/1 -> Vabc/1
  connections:
  Current and Voltage Sensor (Three-Phase)/RConn1 -- PS-Simulink Converter/LConn1
  Current and Voltage Sensor (Three-Phase)/RConn2 -- PS-Simulink Converter1/LConn1
  Current and Voltage Sensor (Three-Phase)/RConn5 -- c/RConn1
  Current and Voltage Sensor (Three-Phase)/RConn4 -- b/RConn1
  Current and Voltage Sensor (Three-Phase)/RConn3 -- a/RConn1
  Current and Voltage Sensor (Three-Phase)/LConn3 -- C/RConn1
  Current and Voltage Sensor (Three-Phase)/LConn1 -- A/RConn1
  Current and Voltage Sensor (Three-Phase)/LConn2 -- B/RConn1

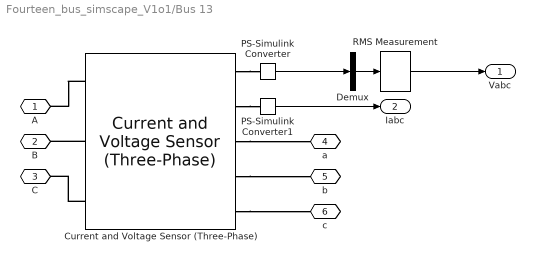
== system Fourteen_bus_simscape_V1o1/Bus 13  ==
  Current and Voltage Sensor (Three-Phase) : ee_lib/Sensors & Transducers/Current and Voltage Sensor (Three-Phase)  port_option=ee.enum.threePhasePort.expanded  vMeasurementType=ee.enum.vmeasurement.ll  outputUnit=ee.enum.unit.si  SRated=100000000 V*A  VRated=0.95 V  I_specify=off  I_priority=None  I=[ 0 0 0 ] A  I_nominal_specify=off  I_nominal_value=1  I_nominal_unit=A  V_specify=off  V_priority=None  V=[ 0 0 0 ] V  V_nominal_specify=off  V_nominal_value=1  V_nominal_unit=V
  Demux : Demux  Outputs=3
  PS-Simulink Converter : nesl_utility/PS-Simulink Converter  PhysicalDomain=network_engine_domain  SubClassName=ps_output  LeftPortType=input  RightPortType=output  PseudoPeriodic=off  Frequencies=[]  VectorFormat=1-D array  Unit=1  AffineConversion=off
  PS-Simulink Converter1 : nesl_utility/PS-Simulink Converter  PhysicalDomain=network_engine_domain  SubClassName=ps_output  LeftPortType=input  RightPortType=output  PseudoPeriodic=off  Frequencies=[]  VectorFormat=1-D array  Unit=1  AffineConversion=off
  RMS Measurement : eeRmsMeasurement/RMS Measurement  LabelModeActiveChoice=Total  F=60  SpecifyHarmonics=off  K=[0 1 2]  Ts=0
      settings: LibrarySourceBlock=|
      | ee_sl_lib/Measurements/RMS
      | Measurement
  A : PMIOPort  Side=Left
  B : PMIOPort  Port=2  Side=Left
  C : PMIOPort  Port=3  Side=Left
  a : PMIOPort  Port=4  Side=Right
  b : PMIOPort  Port=5  Side=Right
  c : PMIOPort  Port=6  Side=Right
  Vabc : Outport  VectorParamsAs1DForOutWhenUnconnected=off
  Iabc : Outport  Port=2  VectorParamsAs1DForOutWhenUnconnected=off
  wires:
  PS-Simulink Converter1/1 -> Iabc/1
  Demux/2 -> RMS Measurement/1
  PS-Simulink Converter/1 -> Demux/1
  RMS Measurement/1 -> Vabc/1
  connections:
  Current and Voltage Sensor (Three-Phase)/RConn1 -- PS-Simulink Converter/LConn1
  Current and Voltage Sensor (Three-Phase)/RConn2 -- PS-Simulink Converter1/LConn1
  Current and Voltage Sensor (Three-Phase)/RConn5 -- c/RConn1
  Current and Voltage Sensor (Three-Phase)/RConn4 -- b/RConn1
  Current and Voltage Sensor (Three-Phase)/RConn3 -- a/RConn1
  Current and Voltage Sensor (Three-Phase)/LConn3 -- C/RConn1
  Current and Voltage Sensor (Three-Phase)/LConn1 -- A/RConn1
  Current and Voltage Sensor (Three-Phase)/LConn2 -- B/RConn1

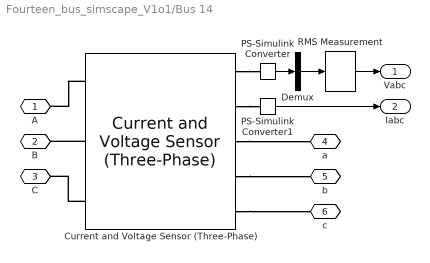
== system Fourteen_bus_simscape_V1o1/Bus 14  ==
  Current and Voltage Sensor (Three-Phase) : ee_lib/Sensors & Transducers/Current and Voltage Sensor (Three-Phase)  port_option=ee.enum.threePhasePort.expanded  vMeasurementType=ee.enum.vmeasurement.ll  outputUnit=ee.enum.unit.si  SRated=100000000 V*A  VRated=0.92 V  I_specify=off  I_priority=None  I=[ 0 0 0 ] A  I_nominal_specify=off  I_nominal_value=1  I_nominal_unit=A  V_specify=off  V_priority=None  V=[ 0 0 0 ] V  V_nominal_specify=off  V_nominal_value=1  V_nominal_unit=V
  Demux : Demux  Outputs=3
  PS-Simulink Converter : nesl_utility/PS-Simulink Converter  PhysicalDomain=network_engine_domain  SubClassName=ps_output  LeftPortType=input  RightPortType=output  PseudoPeriodic=off  Frequencies=[]  VectorFormat=1-D array  Unit=1  AffineConversion=off
  PS-Simulink Converter1 : nesl_utility/PS-Simulink Converter  PhysicalDomain=network_engine_domain  SubClassName=ps_output  LeftPortType=input  RightPortType=output  PseudoPeriodic=off  Frequencies=[]  VectorFormat=1-D array  Unit=1  AffineConversion=off
  RMS Measurement : eeRmsMeasurement/RMS Measurement  LabelModeActiveChoice=Total  F=60  SpecifyHarmonics=off  K=[0 1 2]  Ts=0
      settings: LibrarySourceBlock=|
      | ee_sl_lib/Measurements/RMS
      | Measurement
  A : PMIOPort  Side=Left
  B : PMIOPort  Port=2  Side=Left
  C : PMIOPort  Port=3  Side=Left
  a : PMIOPort  Port=4  Side=Right
  b : PMIOPort  Port=5  Side=Right
  c : PMIOPort  Port=6  Side=Right
  Vabc : Outport  VectorParamsAs1DForOutWhenUnconnected=off
  Iabc : Outport  Port=2  VectorParamsAs1DForOutWhenUnconnected=off
  wires:
  PS-Simulink Converter1/1 -> Iabc/1
  Demux/2 -> RMS Measurement/1
  RMS Measurement/1 -> Vabc/1
  PS-Simulink Converter/1 -> Demux/1
  connections:
  Current and Voltage Sensor (Three-Phase)/RConn1 -- PS-Simulink Converter/LConn1
  Current and Voltage Sensor (Three-Phase)/RConn2 -- PS-Simulink Converter1/LConn1
  Current and Voltage Sensor (Three-Phase)/RConn5 -- c/RConn1
  Current and Voltage Sensor (Three-Phase)/RConn4 -- b/RConn1
  Current and Voltage Sensor (Three-Phase)/RConn3 -- a/RConn1
  Current and Voltage Sensor (Three-Phase)/LConn3 -- C/RConn1
  Current and Voltage Sensor (Three-Phase)/LConn1 -- A/RConn1
  Current and Voltage Sensor (Three-Phase)/LConn2 -- B/RConn1

== system Fourteen_bus_simscape_V1o1/Bus 2  ==
  Current and Voltage Sensor (Three-Phase) : ee_lib/Sensors & Transducers/Current and Voltage Sensor (Three-Phase)  port_option=ee.enum.threePhasePort.expanded  vMeasurementType=ee.enum.vmeasurement.ll  outputUnit=ee.enum.unit.si  SRated=100000000 V*A  VRated=0.95 V  I_specify=off  I_priority=None  I=[ 0 0 0 ] A  I_nominal_specify=off  I_nominal_value=1  I_nominal_unit=A  V_specify=off  V_priority=None  V=[ 0 0 0 ] V  V_nominal_specify=off  V_nominal_value=1  V_nominal_unit=V
  PS-Simulink Converter : nesl_utility/PS-Simulink Converter  PhysicalDomain=network_engine_domain  SubClassName=ps_output  LeftPortType=input  RightPortType=output  PseudoPeriodic=off  Frequencies=[]  VectorFormat=1-D array  Unit=1  AffineConversion=off
  PS-Simulink Converter1 : nesl_utility/PS-Simulink Converter  PhysicalDomain=network_engine_domain  SubClassName=ps_output  LeftPortType=input  RightPortType=output  PseudoPeriodic=off  Frequencies=[]  VectorFormat=1-D array  Unit=1  AffineConversion=off
  A : PMIOPort  Side=Left
  B : PMIOPort  Port=2  Side=Left
  C : PMIOPort  Port=3  Side=Left
  a : PMIOPort  Port=4  Side=Right
  b : PMIOPort  Port=5  Side=Right
  c : PMIOPort  Port=6  Side=Right
  Vabc : Outport  VectorParamsAs1DForOutWhenUnconnected=off
  Iabc : Outport  Port=2  VectorParamsAs1DForOutWhenUnconnected=off
  wires:
  PS-Simulink Converter1/1 -> Iabc/1
  PS-Simulink Converter/1 -> Vabc/1
  connections:
  Current and Voltage Sensor (Three-Phase)/RConn1 -- PS-Simulink Converter/LConn1
  Current and Voltage Sensor (Three-Phase)/RConn2 -- PS-Simulink Converter1/LConn1
  Current and Voltage Sensor (Three-Phase)/RConn5 -- c/RConn1
  Current and Voltage Sensor (Three-Phase)/RConn4 -- b/RConn1
  Current and Voltage Sensor (Three-Phase)/RConn3 -- a/RConn1
  Current and Voltage Sensor (Three-Phase)/LConn3 -- C/RConn1
  Current and Voltage Sensor (Three-Phase)/LConn1 -- A/RConn1
  Current and Voltage Sensor (Three-Phase)/LConn2 -- B/RConn1

== system Fourteen_bus_simscape_V1o1/Bus 3  ==
  Current and Voltage Sensor (Three-Phase) : ee_lib/Sensors & Transducers/Current and Voltage Sensor (Three-Phase)  port_option=ee.enum.threePhasePort.expanded  vMeasurementType=ee.enum.vmeasurement.ll  outputUnit=ee.enum.unit.si  SRated=100000000 V*A  VRated=0.95 V  I_specify=off  I_priority=None  I=[ 0 0 0 ] A  I_nominal_specify=off  I_nominal_value=1  I_nominal_unit=A  V_specify=off  V_priority=None  V=[ 0 0 0 ] V  V_nominal_specify=off  V_nominal_value=1  V_nominal_unit=V
  Demux : Demux  Outputs=3
  PS-Simulink Converter : nesl_utility/PS-Simulink Converter  PhysicalDomain=network_engine_domain  SubClassName=ps_output  LeftPortType=input  RightPortType=output  PseudoPeriodic=off  Frequencies=[]  VectorFormat=1-D array  Unit=1  AffineConversion=off
  PS-Simulink Converter1 : nesl_utility/PS-Simulink Converter  PhysicalDomain=network_engine_domain  SubClassName=ps_output  LeftPortType=input  RightPortType=output  PseudoPeriodic=off  Frequencies=[]  VectorFormat=1-D array  Unit=1  AffineConversion=off
  RMS Measurement : eeRmsMeasurement/RMS Measurement  LabelModeActiveChoice=Total  F=60  SpecifyHarmonics=off  K=[0 1 2]  Ts=0
      settings: LibrarySourceBlock=|
      | ee_sl_lib/Measurements/RMS
      | Measurement
  A : PMIOPort  Side=Left
  B : PMIOPort  Port=2  Side=Left
  C : PMIOPort  Port=3  Side=Left
  a : PMIOPort  Port=4  Side=Right
  b : PMIOPort  Port=5  Side=Right
  c : PMIOPort  Port=6  Side=Right
  Vabc : Outport  VectorParamsAs1DForOutWhenUnconnected=off
  Iabc : Outport  Port=2  VectorParamsAs1DForOutWhenUnconnected=off
  wires:
  PS-Simulink Converter1/1 -> Iabc/1
  RMS Measurement/1 -> Vabc/1
  Demux/1 -> RMS Measurement/1
  PS-Simulink Converter/1 -> Demux/1
  connections:
  Current and Voltage Sensor (Three-Phase)/RConn1 -- PS-Simulink Converter/LConn1
  Current and Voltage Sensor (Three-Phase)/RConn2 -- PS-Simulink Converter1/LConn1
  Current and Voltage Sensor (Three-Phase)/RConn5 -- c/RConn1
  Current and Voltage Sensor (Three-Phase)/RConn4 -- b/RConn1
  Current and Voltage Sensor (Three-Phase)/RConn3 -- a/RConn1
  Current and Voltage Sensor (Three-Phase)/LConn3 -- C/RConn1
  Current and Voltage Sensor (Three-Phase)/LConn1 -- A/RConn1
  Current and Voltage Sensor (Three-Phase)/LConn2 -- B/RConn1

== system Fourteen_bus_simscape_V1o1/Bus 4  ==
  Current and Voltage Sensor (Three-Phase) : ee_lib/Sensors & Transducers/Current and Voltage Sensor (Three-Phase)  port_option=ee.enum.threePhasePort.expanded  vMeasurementType=ee.enum.vmeasurement.ll  outputUnit=ee.enum.unit.si  SRated=100000000 V*A  VRated=0.95 V  I_specify=off  I_priority=None  I=[ 0 0 0 ] A  I_nominal_specify=off  I_nominal_value=1  I_nominal_unit=A  V_specify=off  V_priority=None  V=[ 0 0 0 ] V  V_nominal_specify=off  V_nominal_value=1  V_nominal_unit=V
  Demux : Demux  Outputs=3
  PS-Simulink Converter : nesl_utility/PS-Simulink Converter  PhysicalDomain=network_engine_domain  SubClassName=ps_output  LeftPortType=input  RightPortType=output  PseudoPeriodic=off  Frequencies=[]  VectorFormat=1-D array  Unit=1  AffineConversion=off
  PS-Simulink Converter1 : nesl_utility/PS-Simulink Converter  PhysicalDomain=network_engine_domain  SubClassName=ps_output  LeftPortType=input  RightPortType=output  PseudoPeriodic=off  Frequencies=[]  VectorFormat=1-D array  Unit=1  AffineConversion=off
  RMS Measurement : eeRmsMeasurement/RMS Measurement  LabelModeActiveChoice=Total  F=60  SpecifyHarmonics=off  K=[0 1 2]  Ts=0
      settings: LibrarySourceBlock=|
      | ee_sl_lib/Measurements/RMS
      | Measurement
  A : PMIOPort  Side=Left
  B : PMIOPort  Port=2  Side=Left
  C : PMIOPort  Port=3  Side=Left
  a : PMIOPort  Port=4  Side=Right
  b : PMIOPort  Port=5  Side=Right
  c : PMIOPort  Port=6  Side=Right
  Vabc : Outport  VectorParamsAs1DForOutWhenUnconnected=off
  Iabc : Outport  Port=2  VectorParamsAs1DForOutWhenUnconnected=off
  wires:
  PS-Simulink Converter1/1 -> Iabc/1
  PS-Simulink Converter/1 -> Demux/1
  RMS Measurement/1 -> Vabc/1
  Demux/3 -> RMS Measurement/1
  connections:
  Current and Voltage Sensor (Three-Phase)/RConn1 -- PS-Simulink Converter/LConn1
  Current and Voltage Sensor (Three-Phase)/RConn2 -- PS-Simulink Converter1/LConn1
  Current and Voltage Sensor (Three-Phase)/RConn5 -- c/RConn1
  Current and Voltage Sensor (Three-Phase)/RConn4 -- b/RConn1
  Current and Voltage Sensor (Three-Phase)/RConn3 -- a/RConn1
  Current and Voltage Sensor (Three-Phase)/LConn3 -- C/RConn1
  Current and Voltage Sensor (Three-Phase)/LConn1 -- A/RConn1
  Current and Voltage Sensor (Three-Phase)/LConn2 -- B/RConn1

== system Fourteen_bus_simscape_V1o1/Bus 5  ==
  Current and Voltage Sensor (Three-Phase) : ee_lib/Sensors & Transducers/Current and Voltage Sensor (Three-Phase)  port_option=ee.enum.threePhasePort.expanded  vMeasurementType=ee.enum.vmeasurement.ll  outputUnit=ee.enum.unit.si  SRated=100000000 V*A  VRated=0.95 V  I_specify=off  I_priority=None  I=[ 0 0 0 ] A  I_nominal_specify=off  I_nominal_value=1  I_nominal_unit=A  V_specify=off  V_priority=None  V=[ 0 0 0 ] V  V_nominal_specify=off  V_nominal_value=1  V_nominal_unit=V
  Demux : Demux  Outputs=3
  PS-Simulink Converter : nesl_utility/PS-Simulink Converter  PhysicalDomain=network_engine_domain  SubClassName=ps_output  LeftPortType=input  RightPortType=output  PseudoPeriodic=off  Frequencies=[]  VectorFormat=1-D array  Unit=1  AffineConversion=off
  PS-Simulink Converter1 : nesl_utility/PS-Simulink Converter  PhysicalDomain=network_engine_domain  SubClassName=ps_output  LeftPortType=input  RightPortType=output  PseudoPeriodic=off  Frequencies=[]  VectorFormat=1-D array  Unit=1  AffineConversion=off
  RMS Measurement : eeRmsMeasurement/RMS Measurement  LabelModeActiveChoice=Total  F=60  SpecifyHarmonics=off  K=[0 1 2]  Ts=0
      settings: LibrarySourceBlock=|
      | ee_sl_lib/Measurements/RMS
      | Measurement
  A : PMIOPort  Side=Left
  B : PMIOPort  Port=2  Side=Left
  C : PMIOPort  Port=3  Side=Left
  a : PMIOPort  Port=4  Side=Right
  b : PMIOPort  Port=5  Side=Right
  c : PMIOPort  Port=6  Side=Right
  Vabc : Outport  VectorParamsAs1DForOutWhenUnconnected=off
  Iabc : Outport  Port=2  VectorParamsAs1DForOutWhenUnconnected=off
  wires:
  PS-Simulink Converter1/1 -> Iabc/1
  RMS Measurement/1 -> Vabc/1
  PS-Simulink Converter/1 -> Demux/1
  Demux/2 -> RMS Measurement/1
  connections:
  Current and Voltage Sensor (Three-Phase)/RConn1 -- PS-Simulink Converter/LConn1
  Current and Voltage Sensor (Three-Phase)/RConn2 -- PS-Simulink Converter1/LConn1
  Current and Voltage Sensor (Three-Phase)/RConn5 -- c/RConn1
  Current and Voltage Sensor (Three-Phase)/RConn4 -- b/RConn1
  Current and Voltage Sensor (Three-Phase)/RConn3 -- a/RConn1
  Current and Voltage Sensor (Three-Phase)/LConn3 -- C/RConn1
  Current and Voltage Sensor (Three-Phase)/LConn1 -- A/RConn1
  Current and Voltage Sensor (Three-Phase)/LConn2 -- B/RConn1

== system Fourteen_bus_simscape_V1o1/Bus 6  ==
  Current and Voltage Sensor (Three-Phase) : ee_lib/Sensors & Transducers/Current and Voltage Sensor (Three-Phase)  port_option=ee.enum.threePhasePort.expanded  vMeasurementType=ee.enum.vmeasurement.ll  outputUnit=ee.enum.unit.si  SRated=100000000 V*A  VRated=0.95 V  I_specify=off  I_priority=None  I=[ 0 0 0 ] A  I_nominal_specify=off  I_nominal_value=1  I_nominal_unit=A  V_specify=off  V_priority=None  V=[ 0 0 0 ] V  V_nominal_specify=off  V_nominal_value=1  V_nominal_unit=V
  Demux : Demux  Outputs=3
  PS-Simulink Converter : nesl_utility/PS-Simulink Converter  PhysicalDomain=network_engine_domain  SubClassName=ps_output  LeftPortType=input  RightPortType=output  PseudoPeriodic=off  Frequencies=[]  VectorFormat=1-D array  Unit=1  AffineConversion=off
  PS-Simulink Converter1 : nesl_utility/PS-Simulink Converter  PhysicalDomain=network_engine_domain  SubClassName=ps_output  LeftPortType=input  RightPortType=output  PseudoPeriodic=off  Frequencies=[]  VectorFormat=1-D array  Unit=1  AffineConversion=off
  RMS Measurement : eeRmsMeasurement/RMS Measurement  LabelModeActiveChoice=Total  F=60  SpecifyHarmonics=off  K=[0 1 2]  Ts=0
      settings: LibrarySourceBlock=|
      | ee_sl_lib/Measurements/RMS
      | Measurement
  A : PMIOPort  Side=Left
  B : PMIOPort  Port=2  Side=Left
  C : PMIOPort  Port=3  Side=Left
  a : PMIOPort  Port=4  Side=Right
  b : PMIOPort  Port=5  Side=Right
  c : PMIOPort  Port=6  Side=Right
  Vabc : Outport  VectorParamsAs1DForOutWhenUnconnected=off
  Iabc : Outport  Port=2  VectorParamsAs1DForOutWhenUnconnected=off
  wires:
  PS-Simulink Converter1/1 -> Iabc/1
  RMS Measurement/1 -> Vabc/1
  PS-Simulink Converter/1 -> Demux/1
  Demux/2 -> RMS Measurement/1
  connections:
  Current and Voltage Sensor (Three-Phase)/RConn1 -- PS-Simulink Converter/LConn1
  Current and Voltage Sensor (Three-Phase)/RConn2 -- PS-Simulink Converter1/LConn1
  Current and Voltage Sensor (Three-Phase)/RConn5 -- c/RConn1
  Current and Voltage Sensor (Three-Phase)/RConn4 -- b/RConn1
  Current and Voltage Sensor (Three-Phase)/RConn3 -- a/RConn1
  Current and Voltage Sensor (Three-Phase)/LConn3 -- C/RConn1
  Current and Voltage Sensor (Three-Phase)/LConn1 -- A/RConn1
  Current and Voltage Sensor (Three-Phase)/LConn2 -- B/RConn1
